simulink model "AXU5EV_ADC_Observer"  (R2026b)
settings: Solver=FixedStepDiscrete  StopTime=4e-4  FixedStep=2e-8
libraries: AXU5EV_PL_Algorithm_Library x1
settings Model: Creator=lww  LastModifiedBy=lww

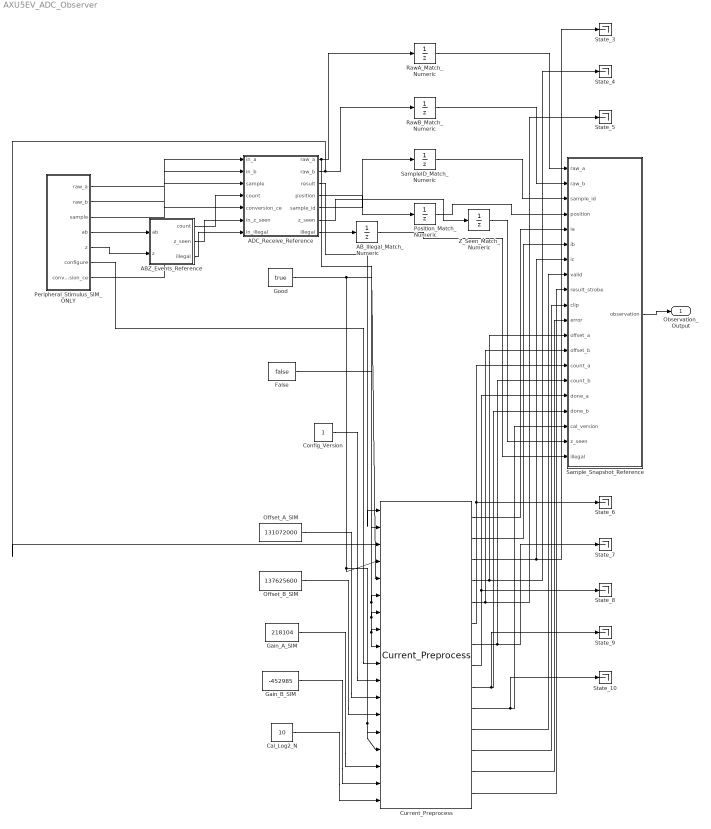
== system AXU5EV_ADC_Observer ==
  ABZ_Events_Reference : MATLAB Function  TreatAsAtomicUnit=on
  AB_Illegal_Match_Numeric : UnitDelay  SampleTime=-1
  ADC_Receive_Reference : MATLAB Function  TreatAsAtomicUnit=on
  Cal_Log2_N : Constant  Value=10  OutDataTypeStr=uint8
  Config_Version : Constant  OutDataTypeStr=uint32
  Current_Preprocess : AXU5EV_PL_Algorithm_Library/Current_Preprocess  SystemSampleTime=-1  VariantActivationTime=update diagram  EmptyChoice=off  PassThrough=off  PassThroughVariantControl=(default)  EmptyChoiceVariantControl=(default)  AllowFlexibleInterface=on  Latency=0  AutoFrameSizeCalculation=off
  False : Constant  Value=false  OutDataTypeStr=boolean
  Gain_A_SIM : Constant  Value=218104  OutDataTypeStr=int32
  Gain_B_SIM : Constant  Value=-452985  OutDataTypeStr=int32
  Good : Constant  Value=true  OutDataTypeStr=boolean
  Offset_A_SIM : Constant  Value=131072000  OutDataTypeStr=int32
  Offset_B_SIM : Constant  Value=137625600  OutDataTypeStr=int32
  Peripheral_Stimulus_SIM_ONLY : MATLAB Function  TreatAsAtomicUnit=on
  Position_Match_Numeric : UnitDelay  SampleTime=-1
  RawA_Match_Numeric : UnitDelay  SampleTime=-1
  RawB_Match_Numeric : UnitDelay  SampleTime=-1
  SampleID_Match_Numeric : UnitDelay  SampleTime=-1
  Sample_Snapshot_Reference : MATLAB Function  TreatAsAtomicUnit=on
  State_{3..10} (8 alike) : Terminator
  Z_Seen_Match_Numeric : UnitDelay  SampleTime=-1
  Observation_Output : Outport  OutDataTypeStr=int64
  wires:
  ADC_Receive_Reference/5(sample_id) -> SampleID_Match_Numeric/1
  ADC_Receive_Reference/4(position) -> Position_Match_Numeric/1
  Peripheral_Stimulus_SIM_ONLY/7(conversion_ce) -> ADC_Receive_Reference/5(conversion_ce)
  ABZ_Events_Reference/1(count) -> ADC_Receive_Reference/4(count)
  Peripheral_Stimulus_SIM_ONLY/5(z) -> ABZ_Events_Reference/2(z)
  Peripheral_Stimulus_SIM_ONLY/4(ab) -> ABZ_Events_Reference/1(ab)
  Peripheral_Stimulus_SIM_ONLY/3(sample) -> ADC_Receive_Reference/3(sample)
  Peripheral_Stimulus_SIM_ONLY/2(raw_b) -> ADC_Receive_Reference/2(in_b)
  Peripheral_Stimulus_SIM_ONLY/1(raw_a) -> ADC_Receive_Reference/1(in_a)
  ABZ_Events_Reference/2(z_seen) -> ADC_Receive_Reference/6(in_z_seen)
  ABZ_Events_Reference/3(illegal) -> ADC_Receive_Reference/7(in_illegal)
  AB_Illegal_Match_Numeric/1 -> Sample_Snapshot_Reference/20(illegal)
  Z_Seen_Match_Numeric/1 -> Sample_Snapshot_Reference/19(z_seen)
  ADC_Receive_Reference/7(illegal) -> AB_Illegal_Match_Numeric/1
  ADC_Receive_Reference/6(z_seen) -> Z_Seen_Match_Numeric/1
  RawA_Match_Numeric/1 -> Sample_Snapshot_Reference/1(raw_a)
  RawB_Match_Numeric/1 -> Sample_Snapshot_Reference/2(raw_b)
  SampleID_Match_Numeric/1 -> Sample_Snapshot_Reference/3(sample_id)
  Position_Match_Numeric/1 -> Sample_Snapshot_Reference/4(position)
  Sample_Snapshot_Reference/1(observation) -> Observation_Output/1
  Current_Preprocess/14 -> Sample_Snapshot_Reference/9(result_strobe)
  Current_Preprocess/13 -> Sample_Snapshot_Reference/11(error)
  Current_Preprocess/12 -> Sample_Snapshot_Reference/10(clip)
  Current_Preprocess/11 -> Sample_Snapshot_Reference/8(valid)
  Current_Preprocess/10 -> Sample_Snapshot_Reference/18(cal_version), State_10/1
  Current_Preprocess/9 -> Sample_Snapshot_Reference/17(done_b), State_9/1
  Current_Preprocess/8 -> Sample_Snapshot_Reference/16(done_a), State_8/1
  Current_Preprocess/7 -> Sample_Snapshot_Reference/15(count_b), State_7/1
  Current_Preprocess/6 -> Sample_Snapshot_Reference/14(count_a), State_6/1
  Current_Preprocess/5 -> Sample_Snapshot_Reference/13(offset_b), State_5/1
  Current_Preprocess/4 -> Sample_Snapshot_Reference/12(offset_a), State_4/1
  Current_Preprocess/3 -> Sample_Snapshot_Reference/7(ic), State_3/1
  Current_Preprocess/2 -> Sample_Snapshot_Reference/6(ib)
  Current_Preprocess/1 -> Sample_Snapshot_Reference/5(ia)
  Cal_Log2_N/1 -> Current_Preprocess/18
  Gain_B_SIM/1 -> Current_Preprocess/17
  Gain_A_SIM/1 -> Current_Preprocess/16
  Offset_B_SIM/1 -> Current_Preprocess/13
  Offset_A_SIM/1 -> Current_Preprocess/12
  Config_Version/1 -> Current_Preprocess/11
  Peripheral_Stimulus_SIM_ONLY/6(configure) -> Current_Preprocess/10
  False/1 -> Current_Preprocess/9, Current_Preprocess/8, Current_Preprocess/7, Current_Preprocess/6
  Good/1 -> Current_Preprocess/15, Current_Preprocess/14, Current_Preprocess/4, Current_Preprocess/5
  ADC_Receive_Reference/3(result) -> Current_Preprocess/1
  ADC_Receive_Reference/1(raw_a) -> Current_Preprocess/2, RawA_Match_Numeric/1
  ADC_Receive_Reference/2(raw_b) -> Current_Preprocess/3, RawB_Match_Numeric/1

== matlab function AXU5EV_ADC_Observer/ADC_Receive_Reference ==
  data: in_a input; raw_a output; in_b input; sample input; count input; raw_b output; result output; position output; sample_id output; conversion_ce input; in_z_seen input; in_illegal input; z_seen output; illegal output
function [raw_a,raw_b,result,position,sample_id,z_seen,illegal]=f(in_a,in_b,sample,count,conversion_ce,in_z_seen,in_illegal)
%#codegen
[raw_a,raw_b,result,position,sample_id,z_seen,illegal]=ax03b1_adc_reference(in_a,in_b,sample,count,conversion_ce,in_z_seen,in_illegal);
end

== matlab function AXU5EV_ADC_Observer/Peripheral_Stimulus_SIM_ONLY ==
  settings: updateMethod=DISCRETE  sampleTime=2e-8
  data: raw_a output; raw_b output; sample output; ab output; z output; configure output; conversion_ce output
function [raw_a,raw_b,sample,ab,z,configure,conversion_ce]=f()
%#codegen
[raw_a,raw_b,sample,ab,z,configure,conversion_ce]=ax03b1_stimulus();
end

== matlab function AXU5EV_ADC_Observer/ABZ_Events_Reference ==
  data: ab input; count output; z input; z_seen output; illegal output
function [count,z_seen,illegal] = f(ab,z)
%#codegen
[count,z_seen,illegal] = ax03b1_abz_reference(ab,z);
end

== matlab function AXU5EV_ADC_Observer/Sample_Snapshot_Reference ==
  data: raw_a input; observation output; raw_b input; sample_id input; position input; ia input; ib input; ic input; valid input; result_strobe input; clip input; error input; offset_a input; offset_b input; count_a input; count_b input; done_a input; done_b input; cal_version input; z_seen input; illegal input
function observation=f(raw_a,raw_b,sample_id,position,ia,ib,ic,valid,result_strobe,clip,error,offset_a,offset_b,count_a,count_b,done_a,done_b,cal_version,z_seen,illegal)
%#codegen
observation=ax03b1_snapshot_reference(raw_a,raw_b,sample_id,position,ia,ib,ic,valid,result_strobe,clip,error,offset_a,offset_b,count_a,count_b,done_a,done_b,cal_version,z_seen,illegal);
end
